simulink model "ASM_Traffic_new"  (R2024a)
settings: Solver=ode1  StartTime=SIM.tstart.v  StopTime=SIM.tend.v  FixedStep=SIM.StepSize.v  RelTol=1e-3
PostLoadFcn:
  | if any(exist('dsrtsu_mdlpostloadfcn', 'file') ~= 0), dsrtsu_mdlpostloadfcn('Execute', bdroot); end
  | try, asm_mdl_postloadfcn(bdroot, 'UpdateModel', 3600); catch, disp(lasterr); end,
InitFcn:
  | , if any(exist('rtifpga_mdlclblib', 'file') ~= 0), rtifpga_mdlclblib('Init', bdroot); end,
  | , if any(exist('dsmpb_private', 'file') ~= 0), dsmpb_private('dsmpb_mdlclblib', 'Init', bdroot); end,
undefined symbols (not defined in the file): _to_, a0b2, ASM_BrakeHydraulics_DemoSystems, ASM_VehicleDynamics_DemoSystems, b98103fe8ad365046cd0, BrakeCircuit, CPT, Crankshaft, DiscIntNeverNeededParam, dsmsi, FinalDriveAssembly, MDL, ModeSignals, Pos_BrakePedal_Maneuver, rad, RefSignals, s_to_rpm, SIM, SoftECU, Suspension, Tire, Transmission
libraries: ASM_Traffic_lib x135, simulink x100, ASM_Utils_lib x77, ASM_VehicleDynamics_lib x70, ASM_Environment_lib x22, dsmpblib x20, dsmsilib x15, MDLD_Utils_lib x10, ASM_BrakeHydraulics_lib x3
(part 44 of 63)

== system ASM_Traffic_new/VehicleDynamics/Plant/VehicleDynamics/Tire/Tire_FR ==
  Coeff_Fric_Road[] : Inport
  " Pos_z_CP_CoorSys_E[m]" : Inport  Port=2
  UnitVec_z_CP_CoorSys_E[x;y;z] : Inport  Port=3
  Pos_Wheels_CoorSys_E[x;y;z][m] : Inport  Port=4
  v_Abs_WheelBody_CoorSys_V[x;y;z][m|s] : Inport  Port=5
  w_Abs_Wheel_CoorSys_V[x;y;z][rad|s] : Inport  Port=6
  RotationMatrix_V_to_E_T[3x3] : Inport  Port=7
  UnitVec_y_Wheel_CoorSys_V[x;y;z] : Inport  Port=8
  omega_Wheel[rad|s] : Inport  Port=9
  Sw_Tire_Parameter_Set[1|2|3|4] : Inport  Port=10
  Reset[] : Inport  Port=11
  Mode[1Normal|2Mirror|3Symmetric] : Inport  Port=12
  p[Pa] : Inport  Port=13
  Tire_Switches : Inport  Port=14
  Bus Selector : BusSelector  OutputSignals=Sw_r_Tire[1:intern;2:extern],r_Tire_extern[m]
  CONTACT_POINT_CALCULATION_FR : ASM_VehicleDynamics_lib/VehicleDynamics/Tire/Base/CONTACT_POINT_CALCULATION  Tag=ASM_SUBCOMPONENT  ASMProperties=struct('Name','CONTACT_POINT_CALCULATION','Version','1.0','Library','ASM_VehicleDynamics_lib')  ASMInstanceName=contact_point_calculation_fr  ASMInstanceID=2
      settings: AttributesFormatString=Instance Name: %<ASMInstanceName>\nInstance ID: %<ASMInstanceID>
  OpenTire : ASM_Utils_lib/Miscellaneous/OpenSystem  popupLibBlk=<select here>  popupTargetDemo=<select here>  Demosystem=VehicleDynamics_Tire  variantLib=ASM_VehicleDynamics_DemoSystems/Tire
  TIRE_FORCES_AND_TORQUES_VECTORS_FR : ASM_VehicleDynamics_lib/VehicleDynamics/Tire/Base/TIRE_FORCES_AND_TORQUES_VECTORS  Tag=ASM_SUBCOMPONENT  ASMProperties=struct('Name','TIRE_FORCES_AND_TORQUES_VECTORS','Version','1.0','Library','ASM_VehicleDynamics_lib')  ASMInstanceName=tire_forces_and_torque_vectors_fr  ASMInstanceID=2
      settings: AttributesFormatString=Instance Name: %<ASMInstanceName>\nInstance ID: %<ASMInstanceID>
  Terminator : Terminator
  Tire_FR : Subsystem  Tag=VehicleDynamics_Tire
  F_Tire[x;y;z][N] : Outport  VectorParamsAs1DForOutWhenUnconnected=off
  Trq_Tire[x;y;z][Nm] : Outport  Port=2  VectorParamsAs1DForOutWhenUnconnected=off
  Trq_Tire_Wheel[Nm] : Outport  Port=3  VectorParamsAs1DForOutWhenUnconnected=off
  Stiffness_z_Tire[N|m] : Outport  Port=4  VectorParamsAs1DForOutWhenUnconnected=off
  tag scope: ASMBUS_VehicleDynamics_Tire_FR_ContactPoint=scoped, ASMBUS_VehicleDynamics_Tire_FR_ForcesAndTorques=scoped, ASMBUS_VehicleDynamics_Tire_FR_Tire=scoped
  wires:
  Sw_Tire_Parameter_Set[1|2|3|4]/1 -> Tire_FR/1(Sw_Tire_Parameter_Set[1|2|3|4])
  Coeff_Fric_Road[]/1 -> Tire_FR/2(Coeff_Fric_Road[])
  omega_Wheel[rad|s]/1 -> Tire_FR/3(omega_Wheel[rad|s])
  UnitVec_y_Wheel_CoorSys_V[x;y;z]/1 -> CONTACT_POINT_CALCULATION_FR/7, TIRE_FORCES_AND_TORQUES_VECTORS_FR/11
  CONTACT_POINT_CALCULATION_FR/2 -> Tire_FR/4(r_Tire[m])
  CONTACT_POINT_CALCULATION_FR/3 -> Tire_FR/5(v_x_Wheel_CoorSys_CP[m|s])
  CONTACT_POINT_CALCULATION_FR/4 -> Tire_FR/6(v_y_Wheel_CoorSys_CP[m|s])
  CONTACT_POINT_CALCULATION_FR/5 -> Tire_FR/7(w_z_Wheel_CoorSys_CP[rad|s])
  CONTACT_POINT_CALCULATION_FR/6 -> Tire_FR/8(Sin_Angle_Alpha_Tire[])
  CONTACT_POINT_CALCULATION_FR/11 -> Terminator/1
  CONTACT_POINT_CALCULATION_FR/7 -> TIRE_FORCES_AND_TORQUES_VECTORS_FR/7
  CONTACT_POINT_CALCULATION_FR/8 -> TIRE_FORCES_AND_TORQUES_VECTORS_FR/8
  CONTACT_POINT_CALCULATION_FR/9 -> TIRE_FORCES_AND_TORQUES_VECTORS_FR/9
  CONTACT_POINT_CALCULATION_FR/10 -> TIRE_FORCES_AND_TORQUES_VECTORS_FR/10
  v_Abs_WheelBody_CoorSys_V[x;y;z][m|s]/1 -> CONTACT_POINT_CALCULATION_FR/1
  w_Abs_Wheel_CoorSys_V[x;y;z][rad|s]/1 -> CONTACT_POINT_CALCULATION_FR/2
  Pos_Wheels_CoorSys_E[x;y;z][m]/1 -> CONTACT_POINT_CALCULATION_FR/3
  " Pos_z_CP_CoorSys_E[m]"/1 -> CONTACT_POINT_CALCULATION_FR/4
  UnitVec_z_CP_CoorSys_E[x;y;z]/1 -> CONTACT_POINT_CALCULATION_FR/5
  RotationMatrix_V_to_E_T[3x3]/1 -> CONTACT_POINT_CALCULATION_FR/6
  CONTACT_POINT_CALCULATION_FR/1 -> [ASMBUS_VehicleDynamics_Tire_FR_ContactPoint]
  Tire_FR/1(ASMSignalBus) -> [ASMBUS_VehicleDynamics_Tire_FR_Tire]
  TIRE_FORCES_AND_TORQUES_VECTORS_FR/1 -> [ASMBUS_VehicleDynamics_Tire_FR_ForcesAndTorques]
  TIRE_FORCES_AND_TORQUES_VECTORS_FR/2 -> F_Tire[x;y;z][N]/1
  TIRE_FORCES_AND_TORQUES_VECTORS_FR/3 -> Trq_Tire[x;y;z][Nm]/1
  TIRE_FORCES_AND_TORQUES_VECTORS_FR/4 -> Trq_Tire_Wheel[Nm]/1
  Reset[]/1 -> Tire_FR/9(Reset[]), CONTACT_POINT_CALCULATION_FR/8
  Tire_FR/8(Stiffness_z_Tire[N|m]) -> Stiffness_z_Tire[N|m]/1
  Tire_FR/2(F_x_Dyn_Tire_CoorSys_CP[N]) -> TIRE_FORCES_AND_TORQUES_VECTORS_FR/1
  Tire_FR/3(F_y_Dyn_Tire_CoorSys_CP[N]) -> TIRE_FORCES_AND_TORQUES_VECTORS_FR/2
  Tire_FR/4(F_z_Dyn_Tire_CoorSys_CP[N]) -> TIRE_FORCES_AND_TORQUES_VECTORS_FR/3
  Tire_FR/5(Trq_x_CoorSys_CP[Nm]) -> TIRE_FORCES_AND_TORQUES_VECTORS_FR/4
  Tire_FR/6(Trq_y_CoorSys_W[Nm]) -> TIRE_FORCES_AND_TORQUES_VECTORS_FR/5
  Tire_FR/7(Trq_z_CoorSys_CP[Nm]) -> TIRE_FORCES_AND_TORQUES_VECTORS_FR/6
  Bus Selector/2 -> Tire_FR/11(r_Tire_External[m])  "<r_Tire_extern[m]>"
  Bus Selector/1 -> Tire_FR/10(Sw_r_Tire[1Int|2Ext])  "<Sw_r_Tire[1:intern;2:extern]>"
  Mode[1Normal|2Mirror|3Symmetric]/1 -> Tire_FR/12(Mode[1Normal;2Mirror;3Symmetric])
  p[Pa]/1 -> Tire_FR/13(p[Pa])
  Tire_Switches/1 -> Bus Selector/1

== system ASM_Traffic_new/VehicleDynamics/Plant/VehicleDynamics/Tire/Tire_RL ==
  Coeff_Fric_Road[] : Inport
  " Pos_z_CP_CoorSys_E[m]" : Inport  Port=2
  UnitVec_z_CP_CoorSys_E[x;y;z] : Inport  Port=3
  Pos_Wheels_CoorSys_E[x;y;z][m] : Inport  Port=4
  v_Abs_WheelBody_CoorSys_V[x;y;z][m|s] : Inport  Port=5
  w_Abs_Wheel_CoorSys_V[x;y;z][rad|s] : Inport  Port=6
  RotationMatrix_V_to_E_T[3x3] : Inport  Port=7
  UnitVec_y_Wheel_CoorSys_V[x;y;z] : Inport  Port=8
  omega_Wheel[rad|s] : Inport  Port=9
  Sw_Tire_Parameter_Set[1|2|3|4] : Inport  Port=10
  Reset[] : Inport  Port=11
  Mode[1Normal|2Mirror|3Symmetric] : Inport  Port=12
  p[Pa] : Inport  Port=13
  Tire_Switches : Inport  Port=14
  Bus Selector : BusSelector  OutputSignals=Sw_r_Tire[1:intern;2:extern],r_Tire_extern[m]
  CONTACT_POINT_CALCULATION_RL : ASM_VehicleDynamics_lib/VehicleDynamics/Tire/Base/CONTACT_POINT_CALCULATION  Tag=ASM_SUBCOMPONENT  ASMProperties=struct('Name','CONTACT_POINT_CALCULATION','Version','1.0','Library','ASM_VehicleDynamics_lib')  ASMInstanceName=contact_point_calculation_rl  ASMInstanceID=3
      settings: AttributesFormatString=Instance Name: %<ASMInstanceName>\nInstance ID: %<ASMInstanceID>
  OpenTire : ASM_Utils_lib/Miscellaneous/OpenSystem  popupLibBlk=<select here>  popupTargetDemo=<select here>  Demosystem=VehicleDynamics_Tire  variantLib=ASM_VehicleDynamics_DemoSystems/Tire
  TIRE_FORCES_AND_TORQUES_VECTORS_RL : ASM_VehicleDynamics_lib/VehicleDynamics/Tire/Base/TIRE_FORCES_AND_TORQUES_VECTORS  Tag=ASM_SUBCOMPONENT  ASMProperties=struct('Name','TIRE_FORCES_AND_TORQUES_VECTORS','Version','1.0','Library','ASM_VehicleDynamics_lib')  ASMInstanceName=tire_forces_and_torque_vectors_rl  ASMInstanceID=3
      settings: AttributesFormatString=Instance Name: %<ASMInstanceName>\nInstance ID: %<ASMInstanceID>
  Terminator : Terminator
  Tire_RL : Subsystem  Tag=VehicleDynamics_Tire
  F_Tire[x;y;z][N] : Outport  VectorParamsAs1DForOutWhenUnconnected=off
  Trq_Tire[x;y;z][Nm] : Outport  Port=2  VectorParamsAs1DForOutWhenUnconnected=off
  Trq_Tire_Wheel[Nm] : Outport  Port=3  VectorParamsAs1DForOutWhenUnconnected=off
  Stiffness_z_Tire[N|m] : Outport  Port=4  VectorParamsAs1DForOutWhenUnconnected=off
  tag scope: ASMBUS_VehicleDynamics_Tire_RL_ContactPoint=scoped, ASMBUS_VehicleDynamics_Tire_RL_ForcesAndTorques=scoped, ASMBUS_VehicleDynamics_Tire_RL_Tire=scoped
  wires:
  Sw_Tire_Parameter_Set[1|2|3|4]/1 -> Tire_RL/1(Sw_Tire_Parameter_Set[1|2|3|4])
  Coeff_Fric_Road[]/1 -> Tire_RL/2(Coeff_Fric_Road[])
  omega_Wheel[rad|s]/1 -> Tire_RL/3(omega_Wheel[rad|s])
  UnitVec_y_Wheel_CoorSys_V[x;y;z]/1 -> CONTACT_POINT_CALCULATION_RL/7, TIRE_FORCES_AND_TORQUES_VECTORS_RL/11
  CONTACT_POINT_CALCULATION_RL/2 -> Tire_RL/4(r_Tire[m])
  CONTACT_POINT_CALCULATION_RL/3 -> Tire_RL/5(v_x_Wheel_CoorSys_CP[m|s])
  CONTACT_POINT_CALCULATION_RL/4 -> Tire_RL/6(v_y_Wheel_CoorSys_CP[m|s])
  CONTACT_POINT_CALCULATION_RL/5 -> Tire_RL/7(w_z_Wheel_CoorSys_CP[rad|s])
  CONTACT_POINT_CALCULATION_RL/6 -> Tire_RL/8(Sin_Angle_Alpha_Tire[])
  CONTACT_POINT_CALCULATION_RL/11 -> Terminator/1
  CONTACT_POINT_CALCULATION_RL/7 -> TIRE_FORCES_AND_TORQUES_VECTORS_RL/7
  CONTACT_POINT_CALCULATION_RL/8 -> TIRE_FORCES_AND_TORQUES_VECTORS_RL/8
  CONTACT_POINT_CALCULATION_RL/9 -> TIRE_FORCES_AND_TORQUES_VECTORS_RL/9
  CONTACT_POINT_CALCULATION_RL/10 -> TIRE_FORCES_AND_TORQUES_VECTORS_RL/10
  v_Abs_WheelBody_CoorSys_V[x;y;z][m|s]/1 -> CONTACT_POINT_CALCULATION_RL/1
  w_Abs_Wheel_CoorSys_V[x;y;z][rad|s]/1 -> CONTACT_POINT_CALCULATION_RL/2
  Pos_Wheels_CoorSys_E[x;y;z][m]/1 -> CONTACT_POINT_CALCULATION_RL/3
  " Pos_z_CP_CoorSys_E[m]"/1 -> CONTACT_POINT_CALCULATION_RL/4
  UnitVec_z_CP_CoorSys_E[x;y;z]/1 -> CONTACT_POINT_CALCULATION_RL/5
  RotationMatrix_V_to_E_T[3x3]/1 -> CONTACT_POINT_CALCULATION_RL/6
  CONTACT_POINT_CALCULATION_RL/1 -> [ASMBUS_VehicleDynamics_Tire_RL_ContactPoint]
  Tire_RL/1(ASMSignalBus) -> [ASMBUS_VehicleDynamics_Tire_RL_Tire]
  TIRE_FORCES_AND_TORQUES_VECTORS_RL/1 -> [ASMBUS_VehicleDynamics_Tire_RL_ForcesAndTorques]
  TIRE_FORCES_AND_TORQUES_VECTORS_RL/2 -> F_Tire[x;y;z][N]/1
  TIRE_FORCES_AND_TORQUES_VECTORS_RL/3 -> Trq_Tire[x;y;z][Nm]/1
  TIRE_FORCES_AND_TORQUES_VECTORS_RL/4 -> Trq_Tire_Wheel[Nm]/1
  Reset[]/1 -> Tire_RL/9(Reset[]), CONTACT_POINT_CALCULATION_RL/8
  Tire_RL/8(Stiffness_z_Tire[N|m]) -> Stiffness_z_Tire[N|m]/1
  Tire_RL/2(F_x_Dyn_Tire_CoorSys_CP[N]) -> TIRE_FORCES_AND_TORQUES_VECTORS_RL/1
  Tire_RL/3(F_y_Dyn_Tire_CoorSys_CP[N]) -> TIRE_FORCES_AND_TORQUES_VECTORS_RL/2
  Tire_RL/4(F_z_Dyn_Tire_CoorSys_CP[N]) -> TIRE_FORCES_AND_TORQUES_VECTORS_RL/3
  Tire_RL/5(Trq_x_CoorSys_CP[Nm]) -> TIRE_FORCES_AND_TORQUES_VECTORS_RL/4
  Tire_RL/6(Trq_y_CoorSys_W[Nm]) -> TIRE_FORCES_AND_TORQUES_VECTORS_RL/5
  Tire_RL/7(Trq_z_CoorSys_CP[Nm]) -> TIRE_FORCES_AND_TORQUES_VECTORS_RL/6
  Bus Selector/2 -> Tire_RL/11(r_Tire_External[m])  "<r_Tire_extern[m]>"
  Bus Selector/1 -> Tire_RL/10(Sw_r_Tire[1Int|2Ext])  "<Sw_r_Tire[1:intern;2:extern]>"
  Mode[1Normal|2Mirror|3Symmetric]/1 -> Tire_RL/12(Mode[1Normal;2Mirror;3Symmetric])
  p[Pa]/1 -> Tire_RL/13(p[Pa])
  Tire_Switches/1 -> Bus Selector/1

== system ASM_Traffic_new/VehicleDynamics/Plant/VehicleDynamics/Tire/Tire_RR ==
  Coeff_Fric_Road[] : Inport
  " Pos_z_CP_CoorSys_E[m]" : Inport  Port=2
  UnitVec_z_CP_CoorSys_E[x;y;z] : Inport  Port=3
  Pos_Wheels_CoorSys_E[x;y;z][m] : Inport  Port=4
  v_Abs_WheelBody_CoorSys_V[x;y;z][m|s] : Inport  Port=5
  w_Abs_Wheel_CoorSys_V[x;y;z][rad|s] : Inport  Port=6
  RotationMatrix_V_to_E_T[3x3] : Inport  Port=7
  UnitVec_y_Wheel_CoorSys_V[x;y;z] : Inport  Port=8
  omega_Wheel[rad|s] : Inport  Port=9
  Sw_Tire_Parameter_Set[1|2|3|4] : Inport  Port=10
  Reset[] : Inport  Port=11
  Mode[1Normal|2Mirror|3Symmetric] : Inport  Port=12
  p[Pa] : Inport  Port=13
  Tire_Switches : Inport  Port=14
  Bus Selector : BusSelector  OutputSignals=Sw_r_Tire[1:intern;2:extern],r_Tire_extern[m]
  CONTACT_POINT_CALCULATION_RR : ASM_VehicleDynamics_lib/VehicleDynamics/Tire/Base/CONTACT_POINT_CALCULATION  Tag=ASM_SUBCOMPONENT  ASMProperties=struct('Name','CONTACT_POINT_CALCULATION','Version','1.0','Library','ASM_VehicleDynamics_lib')  ASMInstanceName=contact_point_calculation_rr  ASMInstanceID=4
      settings: AttributesFormatString=Instance Name: %<ASMInstanceName>\nInstance ID: %<ASMInstanceID>
  OpenTire : ASM_Utils_lib/Miscellaneous/OpenSystem  popupLibBlk=<select here>  popupTargetDemo=<select here>  Demosystem=VehicleDynamics_Tire  variantLib=ASM_VehicleDynamics_DemoSystems/Tire
  TIRE_FORCES_AND_TORQUES_VECTORS_RR : ASM_VehicleDynamics_lib/VehicleDynamics/Tire/Base/TIRE_FORCES_AND_TORQUES_VECTORS  Tag=ASM_SUBCOMPONENT  ASMProperties=struct('Name','TIRE_FORCES_AND_TORQUES_VECTORS','Version','1.0','Library','ASM_VehicleDynamics_lib')  ASMInstanceName=tire_forces_and_torque_vectors_rr  ASMInstanceID=4
      settings: AttributesFormatString=Instance Name: %<ASMInstanceName>\nInstance ID: %<ASMInstanceID>
  Terminator : Terminator
  Tire_RR : Subsystem  Tag=VehicleDynamics_Tire
  F_Tire[x;y;z][N] : Outport  VectorParamsAs1DForOutWhenUnconnected=off
  Trq_Tire[x;y;z][Nm] : Outport  Port=2  VectorParamsAs1DForOutWhenUnconnected=off
  Trq_Tire_Wheel[Nm] : Outport  Port=3  VectorParamsAs1DForOutWhenUnconnected=off
  Stiffness_z_Tire[N|m] : Outport  Port=4  VectorParamsAs1DForOutWhenUnconnected=off
  tag scope: ASMBUS_VehicleDynamics_Tire_RR_ContactPoint=scoped, ASMBUS_VehicleDynamics_Tire_RR_ForcesAndTorques=scoped, ASMBUS_VehicleDynamics_Tire_RR_Tire=scoped
  wires:
  Sw_Tire_Parameter_Set[1|2|3|4]/1 -> Tire_RR/1(Sw_Tire_Parameter_Set[1|2|3|4])
  Coeff_Fric_Road[]/1 -> Tire_RR/2(Coeff_Fric_Road[])
  omega_Wheel[rad|s]/1 -> Tire_RR/3(omega_Wheel[rad|s])
  UnitVec_y_Wheel_CoorSys_V[x;y;z]/1 -> CONTACT_POINT_CALCULATION_RR/7, TIRE_FORCES_AND_TORQUES_VECTORS_RR/11
  CONTACT_POINT_CALCULATION_RR/2 -> Tire_RR/4(r_Tire[m])
  CONTACT_POINT_CALCULATION_RR/3 -> Tire_RR/5(v_x_Wheel_CoorSys_CP[m|s])
  CONTACT_POINT_CALCULATION_RR/4 -> Tire_RR/6(v_y_Wheel_CoorSys_CP[m|s])
  CONTACT_POINT_CALCULATION_RR/5 -> Tire_RR/7(w_z_Wheel_CoorSys_CP[rad|s])
  CONTACT_POINT_CALCULATION_RR/6 -> Tire_RR/8(Sin_Angle_Alpha_Tire[])
  CONTACT_POINT_CALCULATION_RR/11 -> Terminator/1
  CONTACT_POINT_CALCULATION_RR/7 -> TIRE_FORCES_AND_TORQUES_VECTORS_RR/7
  CONTACT_POINT_CALCULATION_RR/8 -> TIRE_FORCES_AND_TORQUES_VECTORS_RR/8
  CONTACT_POINT_CALCULATION_RR/9 -> TIRE_FORCES_AND_TORQUES_VECTORS_RR/9
  CONTACT_POINT_CALCULATION_RR/10 -> TIRE_FORCES_AND_TORQUES_VECTORS_RR/10
  v_Abs_WheelBody_CoorSys_V[x;y;z][m|s]/1 -> CONTACT_POINT_CALCULATION_RR/1
  w_Abs_Wheel_CoorSys_V[x;y;z][rad|s]/1 -> CONTACT_POINT_CALCULATION_RR/2
  Pos_Wheels_CoorSys_E[x;y;z][m]/1 -> CONTACT_POINT_CALCULATION_RR/3
  " Pos_z_CP_CoorSys_E[m]"/1 -> CONTACT_POINT_CALCULATION_RR/4
  UnitVec_z_CP_CoorSys_E[x;y;z]/1 -> CONTACT_POINT_CALCULATION_RR/5
  RotationMatrix_V_to_E_T[3x3]/1 -> CONTACT_POINT_CALCULATION_RR/6
  CONTACT_POINT_CALCULATION_RR/1 -> [ASMBUS_VehicleDynamics_Tire_RR_ContactPoint]
  Tire_RR/1(ASMSignalBus) -> [ASMBUS_VehicleDynamics_Tire_RR_Tire]
  TIRE_FORCES_AND_TORQUES_VECTORS_RR/1 -> [ASMBUS_VehicleDynamics_Tire_RR_ForcesAndTorques]
  TIRE_FORCES_AND_TORQUES_VECTORS_RR/2 -> F_Tire[x;y;z][N]/1
  TIRE_FORCES_AND_TORQUES_VECTORS_RR/3 -> Trq_Tire[x;y;z][Nm]/1
  TIRE_FORCES_AND_TORQUES_VECTORS_RR/4 -> Trq_Tire_Wheel[Nm]/1
  Reset[]/1 -> Tire_RR/9(Reset[]), CONTACT_POINT_CALCULATION_RR/8
  Tire_RR/8(Stiffness_z_Tire[N|m]) -> Stiffness_z_Tire[N|m]/1
  Tire_RR/2(F_x_Dyn_Tire_CoorSys_CP[N]) -> TIRE_FORCES_AND_TORQUES_VECTORS_RR/1
  Tire_RR/3(F_y_Dyn_Tire_CoorSys_CP[N]) -> TIRE_FORCES_AND_TORQUES_VECTORS_RR/2
  Tire_RR/4(F_z_Dyn_Tire_CoorSys_CP[N]) -> TIRE_FORCES_AND_TORQUES_VECTORS_RR/3
  Tire_RR/5(Trq_x_CoorSys_CP[Nm]) -> TIRE_FORCES_AND_TORQUES_VECTORS_RR/4
  Tire_RR/6(Trq_y_CoorSys_W[Nm]) -> TIRE_FORCES_AND_TORQUES_VECTORS_RR/5
  Tire_RR/7(Trq_z_CoorSys_CP[Nm]) -> TIRE_FORCES_AND_TORQUES_VECTORS_RR/6
  Bus Selector/2 -> Tire_RR/11(r_Tire_External[m])  "<r_Tire_extern[m]>"
  Bus Selector/1 -> Tire_RR/10(Sw_r_Tire[1Int|2Ext])  "<Sw_r_Tire[1:intern;2:extern]>"
  Mode[1Normal|2Mirror|3Symmetric]/1 -> Tire_RR/12(Mode[1Normal;2Mirror;3Symmetric])
  p[Pa]/1 -> Tire_RR/13(p[Pa])
  Tire_Switches/1 -> Bus Selector/1

== system ASM_Traffic_new/VehicleDynamics/Plant/VehicleDynamics/VehicleMovement/ASMSignalCollector ==
  Reset[] : Inport
  Vehicle_Movement_Info_Car : Subsystem  mask(VEHICLE_MOVEMENT_INFO_CAR){StepSize=SIM.StepSize}
      mask prompts: StepSize "Simulation Step Size [s]"
      mask help: To collect and calculate typical vehicle data.
  ASMSignalBus : Outport  VectorParamsAs1DForOutWhenUnconnected=off
  wires:
  [ASMBUS_VehicleDynamics_VehicleMotion] -> Vehicle_Movement_Info_Car/4(ASMBUS_VehicleDynamics_VehicleMotion)
  [ASMBUS_VehicleDynamics_CoGAndWheelVelocities] -> Vehicle_Movement_Info_Car/2(CoGAndWheelVelocities)
  [ASMBUS_VehicleDynamics_CoordinateTransformation] -> Vehicle_Movement_Info_Car/3(ASMBUS_VehicleDynamics_CoordinateTransformation)
  Reset[]/1 -> Vehicle_Movement_Info_Car/1(Reset[])
  [ASMBUS_VehicleDynamics_MassForcesAndTorques] -> Vehicle_Movement_Info_Car/5(ASMBUS_VehicleDynamics_MassForcesAndTorques)
  [ASMBUS_VehicleDynamics_VehicleMass] -> Vehicle_Movement_Info_Car/6(ASMBUS_VehicleDynamics_VehicleMass)
  [ASMBUS_VehicleDynamics_SensorMotion] -> Vehicle_Movement_Info_Car/7(ASMBUS_VehicleDynamics_SensorMotion)
  [ASMBUS_VehicleDynamics_Suspension] -> Vehicle_Movement_Info_Car/8(ASMBUS_VehicleDynamics_Suspension)
  Vehicle_Movement_Info_Car/1(ASMSignalBus) -> ASMSignalBus/1
  [ASMBUS_VehicleDynamics_Steering] -> Vehicle_Movement_Info_Car/9(ASMBUS_VehicleDynamics_Steering)

== system ASM_Traffic_new/VehicleDynamics/Plant/VehicleDynamics/VehicleMovement/OR ==
  In1 : Inport
  In2 : Inport  Port=2
  Data Type Conversion : DataTypeConversion  OutDataTypeStr=double  SaturateOnIntegerOverflow=off  RndMeth=Floor
  Logical Operator : Logic  Operator=OR  AllPortsSameDT=off
  Out : Outport  VectorParamsAs1DForOutWhenUnconnected=off
  wires:
  Logical Operator/1 -> Data Type Conversion/1
  In1/1 -> Logical Operator/1
  In2/1 -> Logical Operator/2
  Data Type Conversion/1 -> Out/1

== system ASM_Traffic_new/VehicleDynamics/SignalInterface/ASMSignalInterface/signal_structure/InfoBlock ==

== system ASM_Traffic_new/AnimationInterface/ANIMATION_INTERFACE/Sensors/Object_Sensor_2D_Points/Calc_Object_Sensor_2D_Points/Sensor_Points ==
  Transform_In : Inport
  Angle_Hor_Rel[deg] : Inport  Port=2
  Distance[m] : Inport  Port=3
  Num_SensorRays_Used[] : Inport  Port=4
  Add : Sum
  CheckUnusedPoints : RelationalOperator  Operator=<  OutDataTypeStr=boolean  InputSameDT=off
  Concatenate : Concatenate  NumInputs=3  Mode=Multidimensional array
  Constant1 : Constant  Value=0.99999
  Cos : Trigonometry  Operator=cos
  Deg2Rad : Gain  Gain=pi/180
  Demux : Demux
  Demux1 : Demux
  Demux2 : Demux
  DownAway : Constant  Value=-999999
  ForIterator_Current : Subsystem  TreatAsAtomicUnit=on
  Product{,1..6} (7 alike) : Product
  Reshape : Reshape  OutputDimensionality=Row vector (2-D)
  Reshape1 : Reshape  OutputDimensionality=Row vector (2-D)
  Reshape2 : Reshape  OutputDimensionality=Row vector (2-D)
  Row0 : Selector  NumberOfDimensions=2  IndexMode=Zero-based  InputPortWidth=3  IndexOptions=Index vector (dialog),Index vector (dialog)  Indices=0,-1  OutputSizes=1,1
  Row1 : Selector  NumberOfDimensions=2  IndexMode=Zero-based  InputPortWidth=3  IndexOptions=Index vector (dialog),Index vector (dialog)  Indices=1,-1  OutputSizes=1,1
  Row2 : Selector  NumberOfDimensions=2  IndexMode=Zero-based  InputPortWidth=3  IndexOptions=Index vector (dialog),Index vector (dialog)  Indices=2,-1  OutputSizes=1,1
  Sin : Trigonometry
  Term : Terminator
  Term1 : Terminator
  Term2 : Terminator
  X : Sum  Inputs=+++
  Y : Sum  Inputs=+++
  Z : Sum  Inputs=+++
  dim_animation_point[] : Constant  Value=60
  init_animation_point[] : Constant  Value=zeros(1,60)  VectorParams1D=off
  x1 : Product
  y1 : Product
  y2 : Product
  y3 : Product
  Translate[x;y;z][m] : Outport  VectorParamsAs1DForOutWhenUnconnected=off
  wires:
  y3/1 -> Concatenate/2
  y2/1 -> Concatenate/1
  init_animation_point[]/1 -> ForIterator_Current/2(init_animation_point[])
  Reshape1/1 -> y3/2
  Reshape/1 -> y2/1
  Angle_Hor_Rel[deg]/1 -> ForIterator_Current/5(angle_sensor_out)
  Distance[m]/1 -> ForIterator_Current/4(distance_sensor_out)
  dim_animation_point[]/1 -> ForIterator_Current/1(dim_animation_point[])
  Num_SensorRays_Used[]/1 -> ForIterator_Current/3(num_sensor_rays[])
  ForIterator_Current/2(angle_animation_point[deg]) -> Deg2Rad/1
  Deg2Rad/1 -> Cos/1, Sin/1
  ForIterator_Current/1(distance_animation_point[m]) -> y1/1, x1/1
  Cos/1 -> x1/2
  Sin/1 -> y1/2
  Transform_In/1 -> Row2/1, Row1/1, Row0/1
  x1/1 -> Product5/2, Product6/2, Product4/2, Product2/2
  y1/1 -> Product3/2, Product1/2
  Row0/1 -> Demux/1
  Demux/1 -> Product2/1
  Demux/2 -> Product1/1
  Demux/3 -> Term/1
  Product2/1 -> X/1
  Product1/1 -> X/2
  Demux/4 -> X/3
  Row1/1 -> Demux1/1
  Demux1/1 -> Product4/1
  Demux1/2 -> Product3/1
  Demux1/3 -> Term1/1
  Product4/1 -> Y/1
  Product3/1 -> Y/2
  Demux1/4 -> Y/3
  Concatenate/1 -> Translate[x;y;z][m]/1
  X/1 -> Reshape/1
  Y/1 -> Reshape1/1
  Row2/1 -> Demux2/1
  Demux2/1 -> Product6/1
  Demux2/2 -> Product5/1
  Demux2/3 -> Term2/1
  Product6/1 -> Z/1
  Product5/1 -> Z/2
  Demux2/4 -> Z/3
  Z/1 -> Reshape2/1
  ForIterator_Current/3(flag_point_used[0|1]) -> y2/2, y3/1, CheckUnusedPoints/1
  Reshape2/1 -> Add/2
  Add/1 -> Concatenate/3
  DownAway/1 -> Product/2
  Product/1 -> Add/1
  Constant1/1 -> CheckUnusedPoints/2
  CheckUnusedPoints/1 -> Product/1

== system ASM_Traffic_new/DomainControl/DriverAssistance/Control/SoftECU_ACC/Soft_ECU_ACC/ASMSignalCollector ==
  BusCreator1 : BusCreator  Inputs=4
  ASMSignalBus : Outport  VectorParamsAs1DForOutWhenUnconnected=off
  wires:
  [ASMBUS_SoftECU_ACC_Controller] -> BusCreator1/1
  [ASMBUS_SoftECU_ACC_Interface] -> BusCreator1/2
  BusCreator1/1 -> ASMSignalBus/1  "SoftECU_ACC"
  [ASMBUS_SoftECU_ACC_User_Interface] -> BusCreator1/3
  [ASMBUS_SoftECU_ACC_Target_Selection] -> BusCreator1/4

== system ASM_Traffic_new/DomainControl/DriverAssistance/Control/SoftECU_ACC/Soft_ECU_ACC/ControlModel_Signals ==
  Bus Selector : BusSelector  OutputSignals=ACC_State[1OFF|2Standby|3ON],Driver_Override_ACC_Active[0Off|1On],Driver_Override_ACC_Reason[0NoOverride|1BrakePedal|2AccPedal]
  ACC_State[1OFF|2Standby|3ON] : Outport  VectorParamsAs1DForOutWhenUnconnected=off
  Driver_Override_ACC_Active[0Off|1On] : Outport  Port=2  VectorParamsAs1DForOutWhenUnconnected=off
  Driver_Override_ACC_Reason[0NoOverride|1BrakePedal|2AccPedal] : Outport  Port=3  VectorParamsAs1DForOutWhenUnconnected=off
  wires:
  [ASMBUS_SoftECU_ACC_User_Interface] -> Bus Selector/1
  Bus Selector/1 -> ACC_State[1OFF|2Standby|3ON]/1  "<ACC_State[1OFF|2Standby|3ON]>"
  Bus Selector/2 -> Driver_Override_ACC_Active[0Off|1On]/1  "<Driver_Override_ACC_Active[0Off|1On]>"
  Bus Selector/3 -> Driver_Override_ACC_Reason[0NoOverride|1BrakePedal|2AccPedal]/1  "<Driver_Override_ACC_Reason[0NoOverride|1BrakePedal|2AccPedal]>"

== system ASM_Traffic_new/DomainControl/DriverAssistance/Control/SoftECU_ACC/Soft_ECU_ACC/Input_Selection ==
  PosVec_MainPnt_Fellows[x;y;z][m] : Inport
  Demux : Demux  Outputs=3
  Terminator : Terminator
  Terminator1 : Terminator
  Pos_x_MainPnt_Fellows[m] : Outport  VectorParamsAs1DForOutWhenUnconnected=off
  wires:
  PosVec_MainPnt_Fellows[x;y;z][m]/1 -> Demux/1
  Demux/1 -> Pos_x_MainPnt_Fellows[m]/1
  Demux/2 -> Terminator/1
  Demux/3 -> Terminator1/1

== system ASM_Traffic_new/DomainControl/DriverAssistance/Control/SoftECU_ACC/Soft_ECU_ACC/Map_Inputs ==
  Reset[0|1] : Inport
  Switches_ACC_User : Inport  Port=2
  ECU_Commands[] : Inport  Port=3
  Bus Selector2 : BusSelector  OutputSignals=Sw_ACC_Control_Mode[1ManSched|2Manual],Sw_ACC_On[Off|1On],Sw_ACC_Off[0Off|1On],Sw_ACC_Cancel[0Off|1On],Sw_ACC_Resume[0Off|1On],Sw_ACC_Speed_Set[0Off|1On],Sw_ACC_Speed_Increase[0Off|1On],Sw_ACC_Speed_Decrease[0Off|1On],Sw_ACC_BrakeMode[1Comfort|2AEBOnly|3AEBOff]
  Maneuver : Subsystem
  Multiport Switch{1..8} (8 alike) : MultiPortSwitch  Inputs=2  InputSameDT=off
  Sw_ACC_On[0Off|1On] : Outport  VectorParamsAs1DForOutWhenUnconnected=off
  Sw_ACC_Off[0Off|1On] : Outport  Port=2  VectorParamsAs1DForOutWhenUnconnected=off
  Sw_ACC_Cancel[0Off|1On] : Outport  Port=3  VectorParamsAs1DForOutWhenUnconnected=off
  Sw_ACC_Resume[0Off|1On] : Outport  Port=4  VectorParamsAs1DForOutWhenUnconnected=off
  Sw_ACC_Speed_Set[0Off|1On] : Outport  Port=5  VectorParamsAs1DForOutWhenUnconnected=off
  Sw_ACC_Speed_Increase[0Off|1On] : Outport  Port=6  VectorParamsAs1DForOutWhenUnconnected=off
  Sw_ACC_Speed_Decrease[0Off|1On] : Outport  Port=7  VectorParamsAs1DForOutWhenUnconnected=off
  Sw_ACC_BrakeMode[1Comfort|2AEBOnly|3AEBOff] : Outport  Port=8  VectorParamsAs1DForOutWhenUnconnected=off
  wires:
  Bus Selector2/9 -> Multiport Switch8/3  "<Sw_ACC_BrakeMode[1Comfort|2AEBOnly|3AEBOff]>"
  Maneuver/8(Sw_ACC_BrakeMode[1Comfort|2AEBOnly|3AEBOff]) -> Multiport Switch8/2
  Multiport Switch8/1 -> Sw_ACC_BrakeMode[1Comfort|2AEBOnly|3AEBOff]/1
  Reset[0|1]/1 -> Maneuver/2(Reset[0|1])
  Maneuver/7(Sw_ACC_Speed_Decrease[0Off|1On]) -> Multiport Switch1/2
  Maneuver/6(Sw_ACC_Speed_Increase[0Off|1On]) -> Multiport Switch2/2
  Maneuver/5(Sw_ACC_Speed_Set[0Off|1On]) -> Multiport Switch5/2
  Maneuver/4(Sw_ACC_Resume[0Off|1On]) -> Multiport Switch3/2
  Maneuver/3(Sw_ACC_Cancel[0Off|1On]) -> Multiport Switch4/2
  Maneuver/2(Sw_ACC_Off[0Off|1On]) -> Multiport Switch6/2
  Maneuver/1(Sw_ACC_On[0Off|1On]) -> Multiport Switch7/2
  Bus Selector2/8 -> Multiport Switch1/3  "<Sw_ACC_Speed_Decrease[0Off|1On]>"
  Bus Selector2/7 -> Multiport Switch2/3  "<Sw_ACC_Speed_Increase[0Off|1On]>"
  Bus Selector2/6 -> Multiport Switch5/3  "<Sw_ACC_Speed_Set[0Off|1On]>"
  Bus Selector2/5 -> Multiport Switch3/3  "<Sw_ACC_Resume[0Off|1On]>"
  Bus Selector2/4 -> Multiport Switch4/3  "<Sw_ACC_Cancel[0Off|1On]>"
  Bus Selector2/3 -> Multiport Switch6/3  "<Sw_ACC_Off[0Off|1On]>"
  Bus Selector2/2 -> Multiport Switch7/3  "<Sw_ACC_On[Off|1On]>"
  Bus Selector2/1 -> Multiport Switch1/1, Multiport Switch8/1, Multiport Switch2/1, Multiport Switch5/1, Multiport Switch3/1, Multiport Switch4/1, Multiport Switch6/1, Multiport Switch7/1  "<Sw_ACC_Control_Mode[1ManSched|2Manual]>"
  ECU_Commands[]/1 -> Maneuver/1(ECU_Commands[])
  Switches_ACC_User/1 -> Bus Selector2/1
  Multiport Switch1/1 -> Sw_ACC_Speed_Decrease[0Off|1On]/1
  Multiport Switch2/1 -> Sw_ACC_Speed_Increase[0Off|1On]/1
  Multiport Switch5/1 -> Sw_ACC_Speed_Set[0Off|1On]/1
  Multiport Switch3/1 -> Sw_ACC_Resume[0Off|1On]/1
  Multiport Switch4/1 -> Sw_ACC_Cancel[0Off|1On]/1
  Multiport Switch6/1 -> Sw_ACC_Off[0Off|1On]/1
  Multiport Switch7/1 -> Sw_ACC_On[0Off|1On]/1

== system ASM_Traffic_new/DomainControl/DriverAssistance/Control/SoftECU_ACC/Soft_ECU_ACC/Tire ==
  r_Dyn_Tire[FL;FR;RL;RR][m] : Inport
  Coef_RollingRes[FL;FR;RL;RR][] : Inport  Port=2
  Coef_RolRes_Mean : Fcn  Expr=(u(1)+u(2)+u(3)+u(4))/4
  r_Dyn_Tire_Mean : Fcn  Expr=(u(1)+u(2)+u(3)+u(4))/4
  r_Dyn_Tire_Mean[m] : Outport  VectorParamsAs1DForOutWhenUnconnected=off
  Coef_RollingRes_Mean[] : Outport  Port=2  VectorParamsAs1DForOutWhenUnconnected=off
  wires:
  Coef_RolRes_Mean/1 -> Coef_RollingRes_Mean[]/1
  r_Dyn_Tire_Mean/1 -> r_Dyn_Tire_Mean[m]/1
  r_Dyn_Tire[FL;FR;RL;RR][m]/1 -> r_Dyn_Tire_Mean/1
  Coef_RollingRes[FL;FR;RL;RR][]/1 -> Coef_RolRes_Mean/1

== system ASM_Traffic_new/DomainControl/DriverAssistance/Control/SoftECU_ACC/Soft_ECU_ACC/TrackWidthVehicle ==
  Pos_FL_Wheel[x;y;z][m] : Inport
  Pos_FR_Wheel[x;y;z][m] : Inport  Port=2
  Abs : Abs  SaturateOnIntegerOverflow=off
  Abs1 : Abs  SaturateOnIntegerOverflow=off
  Add : Sum
  Selector : Selector  InputPortWidth=3  IndexOptions=Index vector (dialog)  Indices=[2]  OutputSizes=1
  TrackWidth_Vehicle[m] : Outport  VectorParamsAs1DForOutWhenUnconnected=off
  wires:
  Abs/1 -> Add/1
  Abs1/1 -> Add/2
  Add/1 -> Selector/1
  Selector/1 -> TrackWidth_Vehicle[m]/1
  Pos_FL_Wheel[x;y;z][m]/1 -> Abs/1
  Pos_FR_Wheel[x;y;z][m]/1 -> Abs1/1

== system ASM_Traffic_new/DomainControl/DriverAssistance/Control/SoftECU_ACC/Soft_ECU_ACC/avoid_incomplete_trace2source ==
  In1 : Inport
  DummyGain : Gain
  Out1 : Outport
  wires:
  DummyGain/1 -> Out1/1
  In1/1 -> DummyGain/1

== system ASM_Traffic_new/DomainControl/DriverAssistance/Control/SoftECU_ACC/Soft_ECU_ACC/avoid_incomplete_trace2source1 ==
  In1 : Inport
  DummyGain : Gain
  Out1 : Outport
  wires:
  DummyGain/1 -> Out1/1
  In1/1 -> DummyGain/1

== system ASM_Traffic_new/DomainControl/DriverAssistance/Control/SoftECU_ACC/Soft_ECU_ACC/avoid_incomplete_trace2source10 ==
  In1 : Inport
  DummyGain : Gain
  Out1 : Outport
  wires:
  DummyGain/1 -> Out1/1
  In1/1 -> DummyGain/1

== system ASM_Traffic_new/DomainControl/DriverAssistance/Control/SoftECU_ACC/Soft_ECU_ACC/avoid_incomplete_trace2source2 ==
  In1 : Inport
  DummyGain : Gain
  Out1 : Outport
  wires:
  DummyGain/1 -> Out1/1
  In1/1 -> DummyGain/1

== system ASM_Traffic_new/DomainControl/DriverAssistance/Control/SoftECU_ACC/Soft_ECU_ACC/avoid_incomplete_trace2source4 ==
  In1 : Inport
  DummyGain : Gain
  Out1 : Outport
  wires:
  DummyGain/1 -> Out1/1
  In1/1 -> DummyGain/1

== system ASM_Traffic_new/DomainControl/DriverAssistance/Control/SoftECU_ACC/Soft_ECU_ACC/avoid_incomplete_trace2source5 ==
  In1 : Inport
  DummyGain : Gain
  Out1 : Outport
  wires:
  DummyGain/1 -> Out1/1
  In1/1 -> DummyGain/1

== system ASM_Traffic_new/DomainControl/DriverAssistance/Control/SoftECU_ACC/Soft_ECU_ACC/avoid_incomplete_trace2source6 ==
  In1 : Inport
  DummyGain : Gain
  Out1 : Outport
  wires:
  DummyGain/1 -> Out1/1
  In1/1 -> DummyGain/1

== system ASM_Traffic_new/DomainControl/DriverAssistance/Control/SoftECU_ACC/Soft_ECU_ACC/avoid_incomplete_trace2source7 ==
  In1 : Inport
  DummyGain : Gain
  Out1 : Outport
  wires:
  DummyGain/1 -> Out1/1
  In1/1 -> DummyGain/1

== system ASM_Traffic_new/DomainControl/DriverAssistance/Control/SoftECU_ACC/Soft_ECU_ACC/avoid_incomplete_trace2source8 ==
  In1 : Inport
  DummyGain : Gain
  Out1 : Outport
  wires:
  DummyGain/1 -> Out1/1
  In1/1 -> DummyGain/1

== system ASM_Traffic_new/DomainControl/DriverAssistance/Control/SoftECU_ACC/Soft_ECU_ACC/avoid_incomplete_trace2source9 ==
  In1 : Inport
  DummyGain : Gain
  Out1 : Outport
  wires:
  DummyGain/1 -> Out1/1
  In1/1 -> DummyGain/1

== system ASM_Traffic_new/DomainControl/DriverAssistance/Control/UserInterface/DISP_Control/ACC_Control_Mode[0OFF|1CC|2DC] ==
  In1 : Inport
  Out1 : Outport  VectorParamsAs1DForOutWhenUnconnected=off
  wires:
  In1/1 -> Out1/1

== system ASM_Traffic_new/DomainControl/DriverAssistance/Control/UserInterface/DISP_Control/ACC_State[0OFF|2Standby|3ON] ==
  In1 : Inport
  Out1 : Outport  VectorParamsAs1DForOutWhenUnconnected=off
  wires:
  In1/1 -> Out1/1

== system ASM_Traffic_new/DomainControl/DriverAssistance/Control/UserInterface/DISP_Control/AEB[0Off|1On] ==
  In1 : Inport
  Out1 : Outport  VectorParamsAs1DForOutWhenUnconnected=off
  wires:
  In1/1 -> Out1/1

== system ASM_Traffic_new/DomainControl/DriverAssistance/Control/UserInterface/DISP_Control/Collision[0Off|1On] ==
  In1 : Inport
  Out1 : Outport  VectorParamsAs1DForOutWhenUnconnected=off
  wires:
  In1/1 -> Out1/1

== system ASM_Traffic_new/DomainControl/DriverAssistance/Control/UserInterface/DISP_Control/Control_Mode_ACC[0Off|1CC|2DC] ==
  In1 : Inport
  Out1 : Outport  VectorParamsAs1DForOutWhenUnconnected=off
  wires:
  In1/1 -> Out1/1

== system ASM_Traffic_new/DomainControl/DriverAssistance/Control/UserInterface/DISP_Control/Dist_Long[m] ==
  In1 : Inport
  Out1 : Outport  VectorParamsAs1DForOutWhenUnconnected=off
  wires:
  In1/1 -> Out1/1

== system ASM_Traffic_new/DomainControl/DriverAssistance/Control/UserInterface/DISP_Control/Distance_Set[m] ==
  In1 : Inport
  Out1 : Outport  VectorParamsAs1DForOutWhenUnconnected=off
  wires:
  In1/1 -> Out1/1

== system ASM_Traffic_new/DomainControl/DriverAssistance/Control/UserInterface/DISP_Control/FCW[0Off|1On] ==
  In1 : Inport
  Out1 : Outport  VectorParamsAs1DForOutWhenUnconnected=off
  wires:
  In1/1 -> Out1/1

== system ASM_Traffic_new/DomainControl/DriverAssistance/Control/UserInterface/DISP_Control/State_ACC[0Off|1On] ==
  In1 : Inport
  Out1 : Outport  VectorParamsAs1DForOutWhenUnconnected=off
  wires:
  In1/1 -> Out1/1

== system ASM_Traffic_new/DomainControl/DriverAssistance/Control/UserInterface/DISP_Control/Sw_BrakeMode[1Comfort|2AEBOnly|3AEBOff] ==
  In1 : Inport
  Out1 : Outport  VectorParamsAs1DForOutWhenUnconnected=off
  wires:
  In1/1 -> Out1/1

== system ASM_Traffic_new/DomainControl/DriverAssistance/Control/UserInterface/DISP_Control/TTC[s] ==
  In1 : Inport
  Out1 : Outport  VectorParamsAs1DForOutWhenUnconnected=off
  wires:
  In1/1 -> Out1/1

== system ASM_Traffic_new/DomainControl/DriverAssistance/Control/UserInterface/DISP_Control/Target_Detected[0|1] ==
  In1 : Inport
  Out1 : Outport  VectorParamsAs1DForOutWhenUnconnected=off
  wires:
  In1/1 -> Out1/1

== system ASM_Traffic_new/DomainControl/DriverAssistance/Control/UserInterface/DISP_Control/Trq_Request_Brake_ACC[Nm] ==
  In1 : Inport
  Out1 : Outport  VectorParamsAs1DForOutWhenUnconnected=off
  wires:
  In1/1 -> Out1/1

== system ASM_Traffic_new/DomainControl/DriverAssistance/Control/UserInterface/DISP_Control/Trq_Request_Engine_ACC[Nm] ==
  In1 : Inport
  Out1 : Outport  VectorParamsAs1DForOutWhenUnconnected=off
  wires:
  In1/1 -> Out1/1

== system ASM_Traffic_new/DomainControl/DriverAssistance/Control/UserInterface/DISP_Control/v_Rel[km|h] ==
  In1 : Inport
  Out1 : Outport  VectorParamsAs1DForOutWhenUnconnected=off
  wires:
  In1/1 -> Out1/1

== system ASM_Traffic_new/DomainControl/DriverAssistance/Control/UserInterface/DISP_Control/v_Set[km|h] ==
  In1 : Inport
  Out1 : Outport  VectorParamsAs1DForOutWhenUnconnected=off
  wires:
  In1/1 -> Out1/1

== system ASM_Traffic_new/DomainControl/DriverAssistance/SignalInterface/ASMSignalInterface/signal_structure/InfoBlock ==

== system ASM_Traffic_new/DomainControl/StartSystem/Control/UserInterface/DISP_Control/Flag_NotPressed_Pedal[0|1] ==
  In1 : Inport
  Out1 : Outport  VectorParamsAs1DForOutWhenUnconnected=off
  wires:
  In1/1 -> Out1/1

== system ASM_Traffic_new/DomainControl/StartSystem/Control/UserInterface/DISP_Control/StartStateButtonLogic ==
  note: State LED is overwritten (set to EngRunning) if start button state is being stimulated and a running engine sttate has been reached
  State_StartButton[-2|-1|0|1|2|3] : Inport
  State_Engine[0|1|2|3|4] : Inport  Port=2
  Mode_StartButtonState[1Stim|2SoftECU] : Inport  Port=3
  AND : Logic  IconShape=distinctive  AllPortsSameDT=off  OutDataTypeStr=boolean
  EngRunning : simulink/Logic and Bit Operations/Compare To Constant  relop===  const=3.0  OutDataTypeStr=boolean
  Stim : simulink/Logic and Bit Operations/Compare To Constant  relop===  const=1  OutDataTypeStr=boolean
  Switch : Switch  Criteria=u2 ~= 0  SaturateOnIntegerOverflow=off  InputSameDT=off
  Out1 : Outport  VectorParamsAs1DForOutWhenUnconnected=off
  wires:
  Mode_StartButtonState[1Stim|2SoftECU]/1 -> Stim/1
  EngRunning/1 -> AND/2
  State_StartButton[-2|-1|0|1|2|3]/1 -> Switch/3
  AND/1 -> Switch/2
  Stim/1 -> AND/1
  Switch/1 -> Out1/1
  State_Engine[0|1|2|3|4]/1 -> EngRunning/1, Switch/1

== system ASM_Traffic_new/DomainControl/StartSystem/Control/UserInterface/DISP_Control/State_StartButton[-2NotAuthorized|-1PowerOff|0Acc|1PowerOn|2StarterOn|3EngRunning] ==
  In1 : Inport
  Out1 : Outport  VectorParamsAs1DForOutWhenUnconnected=off
  wires:
  In1/1 -> Out1/1

== system ASM_Traffic_new/DomainControl/StartSystem/Control/UserInterface/DISP_Control/Sw_Ignition[0|1] ==
  In1 : Inport
  Out1 : Outport  VectorParamsAs1DForOutWhenUnconnected=off
  wires:
  In1/1 -> Out1/1

== system ASM_Traffic_new/DomainControl/StartSystem/Control/UserInterface/DISP_Control/Sw_StarterReq[0|1] ==
  In1 : Inport
  Out1 : Outport  VectorParamsAs1DForOutWhenUnconnected=off
  wires:
  In1/1 -> Out1/1

== system ASM_Traffic_new/DomainControl/StartSystem/SignalInterface/ASMSignalInterface/signal_structure/InfoBlock ==

== system ASM_Traffic_new/DomainControl/TorqueManager/SignalInterface/ASMSignalInterface/signal_structure/InfoBlock ==

== system ASM_Traffic_new/Drivetrain/Plant/Drivetrain/Final_Drive_Assembly/ASMSignalCollector/Clutch_4WD ==
  Mode_Drivetrain[1|2|3|4|5] : Inport
  Clutch_4WD : Subsystem
  Dummy_Clutch_4WD : Subsystem
  MultiportSwitch : MultiPortSwitch  Inputs=5  SaturateOnIntegerOverflow=off  InputSameDT=off
  ASMSignalBus : Outport  VectorParamsAs1DForOutWhenUnconnected=off
  wires:
  Clutch_4WD/1(Out) -> MultiportSwitch/5, MultiportSwitch/6
  Mode_Drivetrain[1|2|3|4|5]/1 -> MultiportSwitch/1
  MultiportSwitch/1 -> ASMSignalBus/1  "Clutch_4WD"
  Dummy_Clutch_4WD/1(Out) -> MultiportSwitch/3, MultiportSwitch/4, MultiportSwitch/2

== system ASM_Traffic_new/Drivetrain/Plant/Drivetrain/Final_Drive_Assembly/ASMSignalCollector/Dummy_TGCL4WD_Shaft ==
  BusCreator1 : BusCreator  Inputs=1
  Dummy_Trq_Shaft_TGCL4WD_Shaft[Nm] : Constant  Value=0
  Out : Outport  VectorParamsAs1DForOutWhenUnconnected=off
  wires:
  BusCreator1/1 -> Out/1  "Shaft_TGCL4WD"
  Dummy_Trq_Shaft_TGCL4WD_Shaft[Nm]/1 -> BusCreator1/1  "Trq_TGCL4WD_Shaft[Nm]"

== system ASM_Traffic_new/Drivetrain/Plant/Drivetrain/Final_Drive_Assembly/ASMSignalCollector/FinalDriveRatio ==
  Drivetrain_Mode[1|2|3|4|5] : Inport
  CentralDifferential : Inport  Port=2
  FrontDifferential : Inport  Port=3
  RearDifferential : Inport  Port=4
  Bus Selector : BusSelector  OutputSignals=Const_i_MainReductionGear[]
  Bus Selector1 : BusSelector  OutputSignals=Const_i_MainReductionGear[]
  Bus Selector2 : BusSelector  OutputSignals=Const_i_MainReductionGear[]
  Bus Selector3 : BusSelector  OutputSignals=Const_TrqDistribution[]
  Minus : Sum  Inputs=+-
  One : Constant  OutDataTypeStr=Inherit: Inherit via back propagation
  Product{1..5} (5 alike) : Product  Inputs=**  SaturateOnIntegerOverflow=on  OutDataTypeStr=Inherit: Same as first input
  Sum : Sum  Inputs=++|  SaturateOnIntegerOverflow=on
  Switch : MultiPortSwitch  Inputs=5  InputSameDT=off
  Switch1 : MultiPortSwitch  Inputs=5  InputSameDT=off
  Switch2 : MultiPortSwitch  Inputs=5  InputSameDT=off
  TrqDistri_FrontDrive[] : Constant  OutDataTypeStr=Inherit: Inherit via back propagation
  TrqDistri_RearDrive[] : Constant  Value=0  OutDataTypeStr=Inherit: Inherit via back propagation
  i_FrontDrive[] : Outport  VectorParamsAs1DForOutWhenUnconnected=off
  i_RearDrive[] : Outport  Port=2  VectorParamsAs1DForOutWhenUnconnected=off
  TrqDistri_Front_Rear[0_1] : Outport  Port=3  VectorParamsAs1DForOutWhenUnconnected=off
  i_FinalDrive[] : Outport  Port=4  VectorParamsAs1DForOutWhenUnconnected=off
  wires:
  One/1 -> Minus/1
  Product5/1 -> Switch2/2
  Bus Selector3/1 -> Switch1/2, Minus/2, Product2/1  "<Const_TrqDistribution[]>"
  Product2/1 -> Sum/2
  Switch2/1 -> i_FinalDrive[]/1  "i_FinalDrive[]"
  Minus/1 -> Product4/1
  Product4/1 -> Sum/1
  Bus Selector2/1 -> Product1/2, Product4/2, Switch2/4  "<Const_i_MainReductionGear[]>"
  Sum/1 -> Product5/2
  Bus Selector1/1 -> Switch/5, Product3/2, Switch/6, Product2/2, Switch2/3, Switch2/5, Switch2/6  "<Const_i_MainReductionGear[]>"
  Drivetrain_Mode[1|2|3|4|5]/1 -> Switch/1, Switch1/1, Switch2/1
  TrqDistri_RearDrive[]/1 -> Switch1/4
  TrqDistri_FrontDrive[]/1 -> Switch1/3, Switch1/6, Switch1/5
  CentralDifferential/1 -> Bus Selector/1, Bus Selector3/1
  Switch1/1 -> TrqDistri_Front_Rear[0_1]/1  "TrqDistri_Front_Rear[0_1]"
  Product1/1 -> i_RearDrive[]/1  "i_RearDrive[]"
  Switch/1 -> i_FrontDrive[]/1  "i_FrontDrive[]"
  Product3/1 -> Switch/3, Switch/2, Switch/4
  Bus Selector/1 -> Product1/1, Product5/1, Product3/1  "<Const_i_MainReductionGear[]>"
  RearDifferential/1 -> Bus Selector2/1
  FrontDifferential/1 -> Bus Selector1/1

== system ASM_Traffic_new/Drivetrain/Plant/Drivetrain/Final_Drive_Assembly/ASMSignalCollector/Shaft_CF ==
  Mode_Drivetrain[1|2|3|4|5] : Inport
  Bus Selector1 : BusSelector  OutputSignals=Shaft_CF
  Dummy_CF_Shaft : Subsystem
  MultiportSwitch : MultiPortSwitch  Inputs=5  SaturateOnIntegerOverflow=off  InputSameDT=off
  ASMSignalBus : Outport  VectorParamsAs1DForOutWhenUnconnected=off
  wires:
  Bus Selector1/1 -> MultiportSwitch/4, MultiportSwitch/3, MultiportSwitch/2  "<Shaft_CF>"
  [ASMBUS_Drivetrain_CentralDifferential] -> Bus Selector1/1
  Dummy_CF_Shaft/1(Out) -> MultiportSwitch/5, MultiportSwitch/6
  MultiportSwitch/1 -> ASMSignalBus/1  "Shaft_CF"
  Mode_Drivetrain[1|2|3|4|5]/1 -> MultiportSwitch/1

== system ASM_Traffic_new/Drivetrain/Plant/Drivetrain/Final_Drive_Assembly/ASMSignalCollector/Shaft_CR ==
  Mode_Drivetrain[1|2|3|4|5] : Inport
  Bus Selector1 : BusSelector  OutputSignals=Shaft_CR
  Dummy_CR_Shaft : Subsystem
  MultiportSwitch : MultiPortSwitch  Inputs=5  SaturateOnIntegerOverflow=off  InputSameDT=off
  ASMSignalBus : Outport  VectorParamsAs1DForOutWhenUnconnected=off
  wires:
  [ASMBUS_Drivetrain_CentralDifferential] -> Bus Selector1/1
  Mode_Drivetrain[1|2|3|4|5]/1 -> MultiportSwitch/1
  MultiportSwitch/1 -> ASMSignalBus/1  "Shaft_CR"
  Bus Selector1/1 -> MultiportSwitch/3, MultiportSwitch/4, MultiportSwitch/2  "<Shaft_CR>"
  Dummy_CR_Shaft/1(Out) -> MultiportSwitch/6, MultiportSwitch/5

== system ASM_Traffic_new/Drivetrain/Plant/Drivetrain/Final_Drive_Assembly/ASMSignalCollector/Transfer_Gearbox ==
  Mode_Drivetrain[1|2|3|4|5] : Inport
  Dummy_Transfer_Gearbox : Subsystem
  MultiportSwitch : MultiPortSwitch  Inputs=5  SaturateOnIntegerOverflow=off  InputSameDT=off
  Transfer_Gearbox : Subsystem
  ASMSignalBus : Outport  VectorParamsAs1DForOutWhenUnconnected=off
  wires:
  Transfer_Gearbox/1(Out) -> MultiportSwitch/5, MultiportSwitch/6
  Dummy_Transfer_Gearbox/1(Out) -> MultiportSwitch/2, MultiportSwitch/4, MultiportSwitch/3
  MultiportSwitch/1 -> ASMSignalBus/1  "TransferGearbox"
  Mode_Drivetrain[1|2|3|4|5]/1 -> MultiportSwitch/1

== system ASM_Traffic_new/Drivetrain/Plant/Drivetrain/Final_Drive_Assembly/ASMSignalCollector/Trq_Shafts ==
  Shaft_FL : Inport
  Shaft_FR : Inport  Port=2
  Shaft_RL : Inport  Port=3
  Shaft_RR : Inport  Port=4
  Add : Sum
  Bus Selector : BusSelector  OutputSignals=Trq_FL_Shaft[Nm]
  Bus Selector1 : BusSelector  OutputSignals=Trq_FR_Shaft[Nm]
  Bus Selector2 : BusSelector  OutputSignals=Trq_RL_Shaft[Nm]
  Bus Selector3 : BusSelector  OutputSignals=Trq_RR_Shaft[Nm]
  Mux : Mux
  Trq_Out_Front_Diff[Nm] : Outport  VectorParamsAs1DForOutWhenUnconnected=off
  Trq_Shaft[FL;FR;RL;RR][Nm] : Outport  Port=2  VectorParamsAs1DForOutWhenUnconnected=off
  wires:
  Bus Selector1/1 -> Add/2, Mux/2  "<Trq_FR_Shaft[Nm]>"
  Bus Selector3/1 -> Mux/4  "<Trq_RR_Shaft[Nm]>"
  Mux/1 -> Trq_Shaft[FL;FR;RL;RR][Nm]/1  "Trq_Shaft[FL;FR;RL;RR][Nm]"
  Add/1 -> Trq_Out_Front_Diff[Nm]/1  "Trq_Out_Front_Diff[Nm]"
  Bus Selector/1 -> Add/1, Mux/1  "<Trq_FL_Shaft[Nm]>"
  Bus Selector2/1 -> Mux/3  "<Trq_RL_Shaft[Nm]>"
  Shaft_FL/1 -> Bus Selector/1
  Shaft_FR/1 -> Bus Selector1/1
  Shaft_RL/1 -> Bus Selector2/1
  Shaft_RR/1 -> Bus Selector3/1

== system ASM_Traffic_new/Drivetrain/Plant/Drivetrain/Final_Drive_Assembly/Differentials/SignalSelection ==
  omega_In_CentralDiff[rad|s] : Inport
  omega_In_FrontDiff[rad|s] : Inport  Port=2
  AWD : simulink/Logic and Bit Operations/Compare To Constant  relop===  const=1  OutDataTypeStr=boolean
  FWD : simulink/Logic and Bit Operations/Compare To Constant  relop===  const=2  OutDataTypeStr=boolean
  OR : Logic  Operator=OR  Inputs=3  AllPortsSameDT=off  OutDataTypeStr=boolean
  RWD : simulink/Logic and Bit Operations/Compare To Constant  relop===  const=3  OutDataTypeStr=boolean
  Saturation[1_5] : Saturate  UpperLimit=5  LowerLimit=1
  Switch : Switch  Criteria=u2 ~= 0  SaturateOnIntegerOverflow=off  InputSameDT=off
  omega_In_Diff[rad|s] : Outport  VectorParamsAs1DForOutWhenUnconnected=off
  wires:
  Switch/1 -> omega_In_Diff[rad|s]/1
  omega_In_FrontDiff[rad|s]/1 -> Switch/3
  omega_In_CentralDiff[rad|s]/1 -> Switch/1
  OR/1 -> Switch/2
  AWD/1 -> OR/1
  FWD/1 -> OR/2
  RWD/1 -> OR/3
  Saturation[1_5]/1 -> RWD/1, FWD/1, AWD/1
  [ASMBUS_Drivetrain_Mode] -> Saturation[1_5]/1

== system ASM_Traffic_new/Drivetrain/Plant/Drivetrain/Final_Drive_Assembly/Differentials/Sw_Axle_Driven_FrontDiff ==
  In[] : Inport
  AWD : simulink/Logic and Bit Operations/Compare To Constant  relop===  const=1  OutDataTypeStr=boolean
  DrivenAxle : Constant
  FWD : simulink/Logic and Bit Operations/Compare To Constant  relop===  const=2  OutDataTypeStr=boolean
  OR : Logic  Operator=OR  AllPortsSameDT=off  OutDataTypeStr=boolean
  Switch : Switch  Criteria=u2 ~= 0  SaturateOnIntegerOverflow=off  InputSameDT=off
  UndrivenAxle : Constant  Value=0
  Out[] : Outport  VectorParamsAs1DForOutWhenUnconnected=off
  wires:
  Switch/1 -> Out[]/1
  OR/1 -> Switch/2
  AWD/1 -> OR/1
  FWD/1 -> OR/2
  In[]/1 -> FWD/1, AWD/1
  UndrivenAxle/1 -> Switch/3
  DrivenAxle/1 -> Switch/1

== system ASM_Traffic_new/Drivetrain/Plant/Drivetrain/Final_Drive_Assembly/Differentials/Sw_Axle_Driven_RearDiff ==
  In[] : Inport
  AWD : simulink/Logic and Bit Operations/Compare To Constant  relop===  const=1  OutDataTypeStr=boolean
  DrivenAxle : Constant
  OR : Logic  Operator=OR  AllPortsSameDT=off  OutDataTypeStr=boolean
  RWD : simulink/Logic and Bit Operations/Compare To Constant  relop===  const=3  OutDataTypeStr=boolean
  Switch : Switch  Criteria=u2 ~= 0  SaturateOnIntegerOverflow=off  InputSameDT=off
  UndrivenAxle : Constant  Value=0
  Out[] : Outport  VectorParamsAs1DForOutWhenUnconnected=off
  wires:
  DrivenAxle/1 -> Switch/1
  UndrivenAxle/1 -> Switch/3
  In[]/1 -> AWD/1, RWD/1
  RWD/1 -> OR/2
  AWD/1 -> OR/1
  OR/1 -> Switch/2
  Switch/1 -> Out[]/1

== system ASM_Traffic_new/Drivetrain/Plant/Drivetrain/Final_Drive_Assembly/Differentials/avoid_incomplete_trace2source ==
  In1 : Inport
  DummyGain : Gain
  Out1 : Outport
  wires:
  DummyGain/1 -> Out1/1
  In1/1 -> DummyGain/1

== system ASM_Traffic_new/Drivetrain/Plant/Drivetrain/Final_Drive_Assembly/Differentials/avoid_incomplete_trace2source1 ==
  In1 : Inport
  DummyGain : Gain
  Out1 : Outport
  wires:
  DummyGain/1 -> Out1/1
  In1/1 -> DummyGain/1

== system ASM_Traffic_new/Drivetrain/Plant/Drivetrain/Final_Drive_Assembly/FF4WD_Parts/avoid_incomplete_trace2source ==
  In1 : Inport
  DummyGain : Gain
  Out1 : Outport
  wires:
  DummyGain/1 -> Out1/1
  In1/1 -> DummyGain/1

== system ASM_Traffic_new/Drivetrain/Plant/Drivetrain/Final_Drive_Assembly/FF4WD_Parts/avoid_incomplete_trace2source1 ==
  In1 : Inport
  DummyGain : Gain
  Out1 : Outport
  wires:
  DummyGain/1 -> Out1/1
  In1/1 -> DummyGain/1

== system ASM_Traffic_new/Drivetrain/Plant/Drivetrain/Transmission/AutomaticTransmission/ASMSignalCollector ==
  BusCreator : BusCreator  Inputs=3
  Signal Conversion : SignalConversion  OverrideOpt=off
  ASMSignalBus : Outport  VectorParamsAs1DForOutWhenUnconnected=off
  wires:
  Signal Conversion/1 -> ASMSignalBus/1  "Automatic"
  [ASMBUS_AT_LockUpClutch] -> BusCreator/1
  [ASMBUS_AT_Gearbox] -> BusCreator/2
  BusCreator/1 -> Signal Conversion/1
  [ASMBUS_AT_TorqueConverter] -> BusCreator/3

== system ASM_Traffic_new/Drivetrain/Plant/Drivetrain/Transmission/AutomaticTransmission/Torque_Summation ==
  Trq_Fric[Nm] : Inport
  Trq_Pump[Nm] : Inport  Port=2
  Trq_Turbine[Nm] : Inport  Port=3
  Add : Sum
  Add1 : Sum
  Trq_In_Converter[Nm] : Outport  InitialOutput=0  VectorParamsAs1DForOutWhenUnconnected=off
  Trq_In_Trm[Nm] : Outport  Port=2  InitialOutput=0  VectorParamsAs1DForOutWhenUnconnected=off
  wires:
  Trq_Pump[Nm]/1 -> Add/1
  Trq_Fric[Nm]/1 -> Add/2, Add1/1
  Trq_Turbine[Nm]/1 -> Add1/2
  Add/1 -> Trq_In_Converter[Nm]/1
  Add1/1 -> Trq_In_Trm[Nm]/1

== system ASM_Traffic_new/Drivetrain/Plant/Drivetrain/Transmission/AutomaticTransmission/avoid_incomplete_trace2source ==
  In1 : Inport
  DummyGain : Gain
  Out1 : Outport
  wires:
  DummyGain/1 -> Out1/1
  In1/1 -> DummyGain/1

== system ASM_Traffic_new/Drivetrain/Plant/Drivetrain/Transmission/AutomaticTransmission/avoid_incomplete_trace2source1 ==
  In1 : Inport
  DummyGain : Gain
  Out1 : Outport
  wires:
  DummyGain/1 -> Out1/1
  In1/1 -> DummyGain/1

== system ASM_Traffic_new/Drivetrain/Plant/Drivetrain/Transmission/ManualTransmission/ASMSignalCollector ==
  BusCreator : BusCreator  Inputs=2
  Signal Conversion : SignalConversion  OverrideOpt=off
  ASMSignalBus : Outport  VectorParamsAs1DForOutWhenUnconnected=off
  wires:
  Signal Conversion/1 -> ASMSignalBus/1  "Manual"
  [ASMBUS_MT_Clutch] -> BusCreator/1
  [ASMBUS_MT_Gearbox] -> BusCreator/2
  BusCreator/1 -> Signal Conversion/1

== system ASM_Traffic_new/Drivetrain/Plant/Drivetrain/Transmission/ManualTransmission/avoid_incomplete_trace2source ==
  In1 : Inport
  DummyGain : Gain
  Out1 : Outport
  wires:
  DummyGain/1 -> Out1/1
  In1/1 -> DummyGain/1

== system ASM_Traffic_new/Drivetrain/Plant/Drivetrain/Transmission/ManualTransmission/avoid_incomplete_trace2source1 ==
  In1 : Inport
  DummyGain : Gain
  Out1 : Outport
  wires:
  DummyGain/1 -> Out1/1
  In1/1 -> DummyGain/1

== system ASM_Traffic_new/Drivetrain/Plant/UserInterface/DISP_Plant/ActiveTransmission/Gear[] ==
  In1 : Inport
  Out1 : Outport  VectorParamsAs1DForOutWhenUnconnected=off
  wires:
  In1/1 -> Out1/1

== system ASM_Traffic_new/Drivetrain/Plant/UserInterface/DISP_Plant/ActiveTransmission/Inertia_Trm[kgm2] ==
  In1 : Inport
  Out1 : Outport  VectorParamsAs1DForOutWhenUnconnected=off
  wires:
  In1/1 -> Out1/1
